simulink library "sm_tracked_vehicle_belt_lib"  (R2025a)
settings: Solver=VariableStepAuto  StartTime=0.0  StopTime=10.0  RelTol=1e-3
values from neighbouring files (symbols this model uses):
  s = [0; cumsum(segLen)]    [resampleConvexHull.m]
  tread_ptcld = tread_ptcld_full(tread_ptcld_inds,:)    [sm_tracked_vehicle_belt_param.m]
undefined symbols (not defined in the file or in its folder): roller_clr, tread_clr, tread_h, tread_l, tread_rad, tread_roller_rad, tread_w, tread_xlen, X, Y, Z
libraries: sm_lib x9, Parts_Lib x4, fl_lib x3, nesl_utility x1
Description:
  | Copyright 2026 The MathWorks, Inc.
settings Model: Creator=smiller  LastModifiedBy=smiller

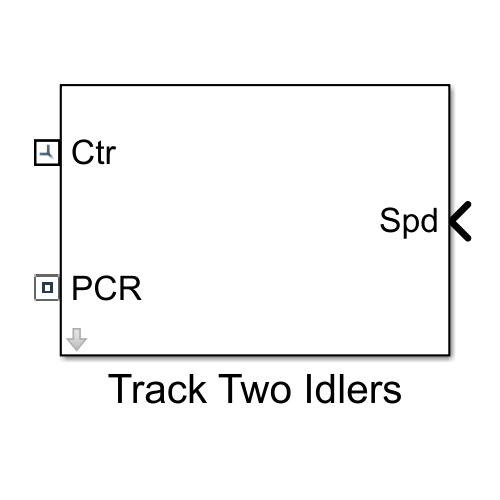
[thumbnail: Simulink's stored preview of the top-level diagram]
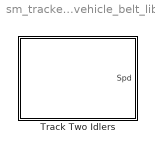
== system sm_tracked_vehicle_belt_lib ==
  Track Two Idlers : Subsystem  mask(Track with Sprocket and 2 Idlers, Point Cloud){cyl_radius=tread_roller_rad, cyl_density=1000, cyl_color_custom=roller_clr, cyl_opacity=1, link_len=tread_l, link_xlen=tread_xlen, link_height=tread_h, link_rado=tread_rad, link_width=tread_w, link_mass=0.5, link_opc=1, link_color=tread_clr, CoordinatesMatrix=tread_ptcld, GraphicSphereRadius=5e-2, GraphicOpacity=1, GraphicDiffuseColor=[0 1 1]}
      mask prompts: cyl_radius "Roller Radius (m)"; cyl_density "Density (kg/m^3)"; cyl_color_custom "Color [R G B] (0-1)"; cyl_opacity "Opacity (0-1)"; link_len "Sprocket-to-Idler (m)"; link_xlen "Center Roller x Position (0-1)"; link_height "Center Roller z Position (m)"; link_rado "Belt Outer Radius (m)"; link_width "Width (m)"; link_mass "Mass (kg)"; link_opc "Opacity (0-1)"; link_color "Color [R G B] (0-1)"; CoordinatesMatrix "Points [x y z] (m)"; GraphicSphereRadius "Radius (m)"; GraphicOpacity "Opacity (0-1)"; GraphicDiffuseColor "Color [R G B] (0-1)"
      mask help: Simple model of a track with one sprocket and 2 idlers.
      mask TypeOptions cyl_radius: Roller F/cyl_radius | Roller H/cyl_radius | Roller R/cyl_radius | Triangle Link/link_radh
      mask TypeOptions cyl_density: Roller F/cyl_density | Roller H/cyl_density | Roller R/cyl_density
      mask TypeOptions cyl_color_custom: Roller F/cyl_color_custom | Roller H/cyl_color_custom | Roller R/cyl_color_custom
      mask TypeOptions cyl_opacity: Roller F/cyl_opacity | Roller H/cyl_opacity | Roller R/cyl_opacity
      mask TypeOptions link_len: Triangle Link/link_len
      mask TypeOptions link_xlen: Triangle Link/link_xlen
      mask TypeOptions link_height: Triangle Link/link_height
      mask TypeOptions link_rado: Triangle Link/link_rado
      mask TypeOptions link_width: Roller F/cyl_length | Roller H/cyl_length | Roller R/cyl_length | Triangle Link/link_thickness
      mask TypeOptions link_mass: Triangle Link/link_mass
      mask TypeOptions link_opc: Triangle Link/link_opc
      mask TypeOptions link_color: Triangle Link/link_color
      mask TypeOptions CoordinatesMatrix: Point Cloud/CoordinatesMatrix
      mask TypeOptions GraphicSphereRadius: Point Cloud/GraphicSphereRadius
      mask TypeOptions GraphicOpacity: Point Cloud/GraphicOpacity
      mask TypeOptions GraphicDiffuseColor: Point Cloud/GraphicDiffuseColor
      mask DialogControl Container4 Prompt: Track
      mask DialogControl Container5 Prompt: Roller
      mask DialogControl Container6 Prompt: Belt
      mask DialogControl Container7 Prompt: Point Cloud

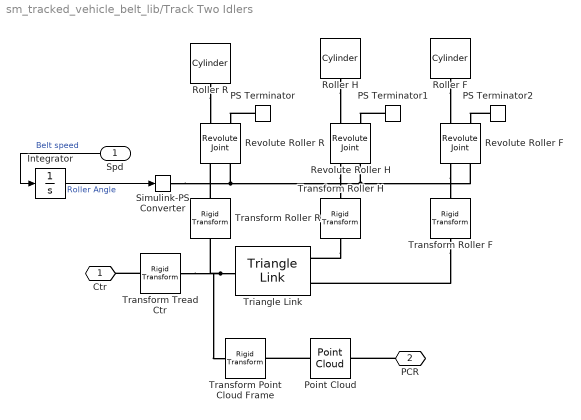
== system sm_tracked_vehicle_belt_lib/Track Two Idlers ==
  Spd : Inport
  Integrator : Integrator
  PS Terminator : fl_lib/Physical Signals/Sinks/PS Terminator
  PS Terminator1 : fl_lib/Physical Signals/Sinks/PS Terminator
  PS Terminator2 : fl_lib/Physical Signals/Sinks/PS Terminator
  Point Cloud : sm_lib/Curves and Surfaces/Point Cloud  CoordinatesMatrix=CoordinatesMatrix  CoordinatesMatrixUnits=m  GraphicType=MarkerCloud  GraphicSphereRadius=GraphicSphereRadius  GraphicSphereRadiusUnits=m  GraphicVisPropType=SimpleVisualProperties  GraphicDiffuseColor=GraphicDiffuseColor  GraphicOpacity=GraphicOpacity  GraphicSpecularColor=[0.5 0.5 0.5 1.0]  GraphicAmbientColor=[0.15 0.15 0.15 1.0]  GraphicEmissiveColor=[0.0 0.0 0.0 1.0]  GraphicShininess=75
  Revolute Roller F : sm_lib/Joints/Revolute Joint  JointMode=Normal  CompositeWrenchDir=FollowerOnBase  CompositeWrenchFrame=BaseFrame  SenseConstraintForce=off  SenseConstraintTorque=off  SenseTotalForce=off  SenseTotalTorque=off  PositionTargetSpecify=off  PositionTargetPriority=High  PositionTargetValue=0  PositionTargetValueUnits=deg  VelocityTargetSpecify=off  VelocityTargetPriority=High  VelocityTargetValue=0  VelocityTargetValueUnits=deg/s  EquilibriumPosition=0  EquilibriumPositionUnits=deg  SpringStiffness=0  SpringStiffnessUnits=N*m/deg  DampingCoefficient=0  DampingCoefficientUnits=N*m/(deg/s)  LowerLimitSpecify=off  LowerLimitBound=-90  LowerLimitBoundUnits=deg  LowerLimitStiffness=1e4  LowerLimitStiffnessUnits=N*m/deg  LowerLimitDamping=10  LowerLimitDampingUnits=N*m/(deg/s)  LowerLimitTransitionRegionWidth=0.1  LowerLimitTransitionRegionWidthUnits=deg  UpperLimitSpecify=off  UpperLimitBound=90  UpperLimitBoundUnits=deg  UpperLimitStiffness=1e4  UpperLimitStiffnessUnits=N*m/deg  UpperLimitDamping=10  UpperLimitDampingUnits=N*m/(deg/s)  UpperLimitTransitionRegionWidth=0.1  UpperLimitTransitionRegionWidthUnits=deg  TorqueActuationMode=ComputedTorque  MotionActuationMode=InputMotion  SensePosition=off  SenseVelocity=off  SenseAcceleration=off  SenseTorqueForce=on  SenseLowerLimitTorqueForce=off  SenseUpperLimitTorqueForce=off
  Revolute Roller H : sm_lib/Joints/Revolute Joint  JointMode=Normal  CompositeWrenchDir=FollowerOnBase  CompositeWrenchFrame=BaseFrame  SenseConstraintForce=off  SenseConstraintTorque=off  SenseTotalForce=off  SenseTotalTorque=off  PositionTargetSpecify=off  PositionTargetPriority=High  PositionTargetValue=0  PositionTargetValueUnits=deg  VelocityTargetSpecify=off  VelocityTargetPriority=High  VelocityTargetValue=0  VelocityTargetValueUnits=deg/s  EquilibriumPosition=0  EquilibriumPositionUnits=deg  SpringStiffness=0  SpringStiffnessUnits=N*m/deg  DampingCoefficient=0  DampingCoefficientUnits=N*m/(deg/s)  LowerLimitSpecify=off  LowerLimitBound=-90  LowerLimitBoundUnits=deg  LowerLimitStiffness=1e4  LowerLimitStiffnessUnits=N*m/deg  LowerLimitDamping=10  LowerLimitDampingUnits=N*m/(deg/s)  LowerLimitTransitionRegionWidth=0.1  LowerLimitTransitionRegionWidthUnits=deg  UpperLimitSpecify=off  UpperLimitBound=90  UpperLimitBoundUnits=deg  UpperLimitStiffness=1e4  UpperLimitStiffnessUnits=N*m/deg  UpperLimitDamping=10  UpperLimitDampingUnits=N*m/(deg/s)  UpperLimitTransitionRegionWidth=0.1  UpperLimitTransitionRegionWidthUnits=deg  TorqueActuationMode=ComputedTorque  MotionActuationMode=InputMotion  SensePosition=off  SenseVelocity=off  SenseAcceleration=off  SenseTorqueForce=on  SenseLowerLimitTorqueForce=off  SenseUpperLimitTorqueForce=off
  Revolute Roller R : sm_lib/Joints/Revolute Joint  JointMode=Normal  CompositeWrenchDir=FollowerOnBase  CompositeWrenchFrame=BaseFrame  SenseConstraintForce=off  SenseConstraintTorque=off  SenseTotalForce=off  SenseTotalTorque=off  PositionTargetSpecify=off  PositionTargetPriority=High  PositionTargetValue=0  PositionTargetValueUnits=deg  VelocityTargetSpecify=off  VelocityTargetPriority=High  VelocityTargetValue=0  VelocityTargetValueUnits=deg/s  EquilibriumPosition=0  EquilibriumPositionUnits=deg  SpringStiffness=0  SpringStiffnessUnits=N*m/deg  DampingCoefficient=0  DampingCoefficientUnits=N*m/(deg/s)  LowerLimitSpecify=off  LowerLimitBound=-90  LowerLimitBoundUnits=deg  LowerLimitStiffness=1e4  LowerLimitStiffnessUnits=N*m/deg  LowerLimitDamping=10  LowerLimitDampingUnits=N*m/(deg/s)  LowerLimitTransitionRegionWidth=0.1  LowerLimitTransitionRegionWidthUnits=deg  UpperLimitSpecify=off  UpperLimitBound=90  UpperLimitBoundUnits=deg  UpperLimitStiffness=1e4  UpperLimitStiffnessUnits=N*m/deg  UpperLimitDamping=10  UpperLimitDampingUnits=N*m/(deg/s)  UpperLimitTransitionRegionWidth=0.1  UpperLimitTransitionRegionWidthUnits=deg  TorqueActuationMode=ComputedTorque  MotionActuationMode=InputMotion  SensePosition=off  SenseVelocity=off  SenseAcceleration=off  SenseTorqueForce=on  SenseLowerLimitTorqueForce=off  SenseUpperLimitTorqueForce=off
  Roller F : Parts_Lib/Cylinder  Tag=CustomStyle  cyl_radius=cyl_radius  cyl_length=link_width  cyl_density=cyl_density  cyl_color=custom  cyl_opacity=cyl_opacity  cyl_color_custom=cyl_color_custom  mark_radius=[0.75 0.5]  mark_len_factor=1.01  mark_angle=60  mark_color=black  mark_opacity=1
  Roller H : Parts_Lib/Cylinder  Tag=CustomStyle  cyl_radius=cyl_radius  cyl_length=link_width  cyl_density=cyl_density  cyl_color=custom  cyl_opacity=cyl_opacity  cyl_color_custom=cyl_color_custom  mark_radius=[0.75 0.5]  mark_len_factor=1.01  mark_angle=60  mark_color=black  mark_opacity=1
  Roller R : Parts_Lib/Cylinder  Tag=CustomStyle  cyl_radius=cyl_radius  cyl_length=link_width  cyl_density=cyl_density  cyl_color=custom  cyl_opacity=cyl_opacity  cyl_color_custom=cyl_color_custom  mark_radius=[0.75 0.5]  mark_len_factor=1.01  mark_angle=60  mark_color=black  mark_opacity=1
  Simulink-PS Converter : nesl_utility/Simulink-PS Converter  PhysicalDomain=network_engine_domain  SubClassName=ps_input  LeftPortType=input  RightPortType=output  PseudoPeriodic=off  Frequencies=[]  NoiseDistribution=none  NoiseParameters=[]  Unit=1  AffineConversion=off  FilteringAndDerivatives=filter  SimscapeFilterOrder=2  InputFilterTimeConstant=0.005  UdotUserProvided=0
  Transform Point Cloud Frame : sm_lib/Frames and Transforms/Rigid Transform  RotationMethod=StandardAxis  FollAlignAxisA=+X  BaseAlignAxisA=+Y  FollAlignAxisB=+Y  BaseAlignAxisB=+Z  RotationStandardAxis=+X  RotationAngle=-90  RotationAngleUnits=deg  RotationArbitraryAxis=[0 0 1]  RotationSequenceAxes=FollowerAxes  RotationSequence=XYX  RotationSequenceAngles=[0 0 0]  RotationSequenceAnglesUnits=deg  RotationMatrix=[1 0 0;0 1 0;0 0 1]  Quaternion=[1 0 0 0]  TranslationMethod=None  TranslationCartesianOffset=[0 0 0]  TranslationCartesianOffsetUnits=m  TranslationStandardAxis=+Z  TranslationStandardOffset=0  TranslationStandardOffsetUnits=m  TranslationROffset=0  TranslationROffsetUnits=m  TranslationThetaOffset=0  TranslationThetaOffsetUnits=deg  TranslationZOffset=0  TranslationZOffsetUnits=m
  Transform Roller F : sm_lib/Frames and Transforms/Rigid Transform  RotationMethod=StandardAxis  FollAlignAxisA=+X  BaseAlignAxisA=+Y  FollAlignAxisB=+Y  BaseAlignAxisB=+Z  RotationStandardAxis=+Y  RotationAngle=180  RotationAngleUnits=deg  RotationArbitraryAxis=[0 0 1]  RotationSequenceAxes=FollowerAxes  RotationSequence=XYX  RotationSequenceAngles=[0 0 0]  RotationSequenceAnglesUnits=deg  RotationMatrix=[1 0 0; 0 1 0; 0 0 1]  Quaternion=[1 0 0 0]  TranslationMethod=None  TranslationCartesianOffset=[0 0 0]  TranslationCartesianOffsetUnits=m  TranslationStandardAxis=+Z  TranslationStandardOffset=0  TranslationStandardOffsetUnits=m  TranslationROffset=0  TranslationROffsetUnits=m  TranslationThetaOffset=0  TranslationThetaOffsetUnits=deg  TranslationZOffset=0  TranslationZOffsetUnits=m
  Transform Roller H : sm_lib/Frames and Transforms/Rigid Transform  RotationMethod=StandardAxis  FollAlignAxisA=+X  BaseAlignAxisA=+Y  FollAlignAxisB=+Y  BaseAlignAxisB=+Z  RotationStandardAxis=+Y  RotationAngle=180  RotationAngleUnits=deg  RotationArbitraryAxis=[0 0 1]  RotationSequenceAxes=FollowerAxes  RotationSequence=XYX  RotationSequenceAngles=[0 0 0]  RotationSequenceAnglesUnits=deg  RotationMatrix=[1 0 0; 0 1 0; 0 0 1]  Quaternion=[1 0 0 0]  TranslationMethod=None  TranslationCartesianOffset=[0 0 0]  TranslationCartesianOffsetUnits=m  TranslationStandardAxis=+Z  TranslationStandardOffset=0  TranslationStandardOffsetUnits=m  TranslationROffset=0  TranslationROffsetUnits=m  TranslationThetaOffset=0  TranslationThetaOffsetUnits=deg  TranslationZOffset=0  TranslationZOffsetUnits=m
  Transform Roller R : sm_lib/Frames and Transforms/Rigid Transform  RotationMethod=StandardAxis  FollAlignAxisA=+X  BaseAlignAxisA=+Y  FollAlignAxisB=+Y  BaseAlignAxisB=+Z  RotationStandardAxis=+Y  RotationAngle=180  RotationAngleUnits=deg  RotationArbitraryAxis=[0 0 1]  RotationSequenceAxes=FollowerAxes  RotationSequence=XYX  RotationSequenceAngles=[0 0 0]  RotationSequenceAnglesUnits=deg  RotationMatrix=[1 0 0; 0 1 0; 0 0 1]  Quaternion=[1 0 0 0]  TranslationMethod=None  TranslationCartesianOffset=[0 0 0]  TranslationCartesianOffsetUnits=m  TranslationStandardAxis=+Z  TranslationStandardOffset=0  TranslationStandardOffsetUnits=m  TranslationROffset=0  TranslationROffsetUnits=m  TranslationThetaOffset=0  TranslationThetaOffsetUnits=deg  TranslationZOffset=0  TranslationZOffsetUnits=m
  Transform Tread Ctr : sm_lib/Frames and Transforms/Rigid Transform  RotationMethod=StandardAxis  FollAlignAxisA=+X  BaseAlignAxisA=+Y  FollAlignAxisB=+Y  BaseAlignAxisB=+Z  RotationStandardAxis=+X  RotationAngle=-90  RotationAngleUnits=deg  RotationArbitraryAxis=[0 0 1]  RotationSequenceAxes=FollowerAxes  RotationSequence=XYX  RotationSequenceAngles=[0 0 0]  RotationSequenceAnglesUnits=deg  RotationMatrix=[1 0 0; 0 1 0; 0 0 1]  Quaternion=[1 0 0 0]  TranslationMethod=StandardAxis  TranslationCartesianOffset=[0 0 0]  TranslationCartesianOffsetUnits=m  TranslationStandardAxis=+X  TranslationStandardOffset=link_len/2  TranslationStandardOffsetUnits=m  TranslationROffset=0  TranslationROffsetUnits=m  TranslationThetaOffset=0  TranslationThetaOffsetUnits=deg  TranslationZOffset=0  TranslationZOffsetUnits=m
  Triangle Link : Parts_Lib/Triangle Link  link_len=link_len  link_height=link_height  link_xlen=link_xlen  link_radh=cyl_radius  link_rado=link_rado  link_thickness=link_width  link_mass=link_mass  link_color=link_color  link_opc=link_opc
  Ctr : PMIOPort  Side=Right
  PCR : PMIOPort  Port=2  Side=Right
  wires:
  Integrator/1 -> Simulink-PS Converter/1  "Roller Angle"
  Spd/1 -> Integrator/1  "Belt speed"
  connections:
  PS Terminator1/LConn1 -- Revolute Roller H/RConn2
  Simulink-PS Converter/RConn1 -- Revolute Roller R/LConn2 -- Revolute Roller F/LConn2 -- Revolute Roller H/LConn2
  Transform Tread Ctr/RConn1 -- Ctr/RConn1
  Transform Roller F/LConn1 -- Triangle Link/RConn2
  Roller F/LConn1 -- Revolute Roller F/RConn1
  Roller H/LConn1 -- Revolute Roller H/RConn1
  Roller R/LConn1 -- Revolute Roller R/RConn1
  Transform Roller H/LConn1 -- Triangle Link/RConn1
  PS Terminator/LConn1 -- Revolute Roller R/RConn2
  PS Terminator2/LConn1 -- Revolute Roller F/RConn2
  Revolute Roller F/LConn1 -- Transform Roller F/RConn1
  Revolute Roller H/LConn1 -- Transform Roller H/RConn1
  Triangle Link/LConn1 -- Transform Tread Ctr/LConn1 -- Transform Roller R/LConn1 -- Transform Point Cloud Frame/LConn1
  Transform Roller R/RConn1 -- Revolute Roller R/LConn1
  PCR/RConn1 -- Point Cloud/RConn1
  Point Cloud/LConn1 -- Transform Point Cloud Frame/RConn1
